simulink model "HexaMotor_LeadLag_Control_V03"  (R2026b)
settings: Solver=FixedStepDiscrete  StopTime=30  FixedStep=0.001  EnableMultiTasking=on
PreLoadFcn:
  | % HexaMotor custom Uno R4 blocks (Encoder Velocity, PWM, Analog Input) are
  | % System objects in the HexaMotorBlocks folder next to this model. Add it to
  | % the path if they aren't found (install_HexaMotor_V03 adds it permanently).
  | if ~exist('R4PWM', 'class') || ~exist('EncoderVelocity', 'class')
  |     addpath(fullfile(fileparts(get_param(bdroot, 'FileName')), 'HexaMotorBlocks'));
  |     if ~exist('R4PWM', 'class')
  |         warning('HexaMotor blocks not found. Run install_HexaMotor_V03 in the HexaMotor folder.');
  |     end
  | end
model workspace (MAT data in the model file):
  sampleRate = 0.001
libraries: simulink x2, eeGeneralControl x2, arduinolib x2, slpidlib x1
settings Model: SILPILModeSetting=veronly  Creator=bkhusain  LastModifiedBy=arkad
settings SolverCC: AutoInsertRateTranBlk=on
settings DataIOCC: DSMLogging=off  ReturnWorkspaceOutputs=off  SaveOutput=off  SaveTime=off
settings OptimizationCC: DifferentSizesBufferReuse=on  EnhancedBackFolding=on  MaxStackSize=64  OptimizationCustomize=off  OptimizeBlockOrder=speed
settings DebuggingCC: ParameterOverflowMsg=none  ParameterPrecisionLossMsg=none  ParameterTunabilityLossMsg=error  ParameterUnderflowMsg=error
settings HardwareCC: ProdHWDeviceType=ARM Compatible->ARM Cortex  ProdLargestAtomicFloat=Double  ProdLargestAtomicInteger=Long
settings SFSimCC: MATLABDynamicMemAlloc=off
settings RTWCC: BuildConfiguration=Faster Runs  DLArmComputeVersion=19.05  Description=Embedded Coder  HardwareBoard=Arduino Uno R4 Minima  SystemTargetFile=ert.tlc  TLCOptions=-aInlineSetEventsForThisBaseRateFcn=TLC_FALSE -aSuppressMultiTaskScheduler=TLC_FALSE -aRateBasedStepFcn=1  TemplateMakefile=ert_default_tmf  Toolchain=Arduino ARM M4
settings CodeAppCC: ForceParamTrailComments=on  OperatorAnnotations=on
settings ERTTargetCC: DynamicArrayContainerType=coder::array  ERTCustomFileBanners=off  ExtModeAutomaticAllocSize=off  ExtModeIntrfLevel=Level2 - Open  ExtModeMexFile=ext_xcp  ExtModeStaticAlloc=on  ModelStepFunctionPrototypeControlCompliant=off  SupportContinuousTime=on  SupportNonInlinedSFcns=on  SupportVariableSizeSignals=on
settings SimscapeCC: SimscapeUseEnergyAccounting=off

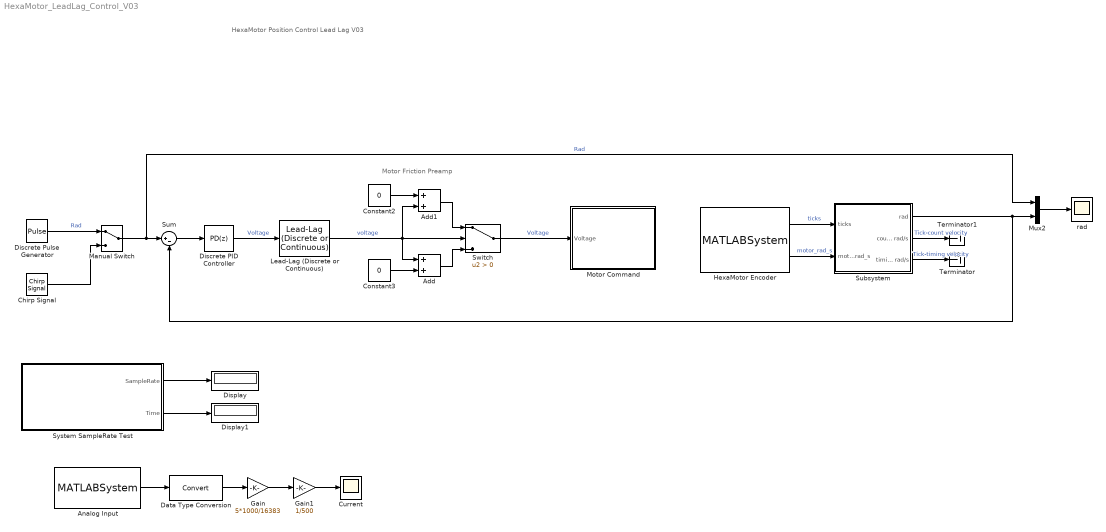
== system HexaMotor_LeadLag_Control_V03 ==
  note: HexaMotor
      | Position Control Lead Lag V03
  note: Motor Friction Preamp
  Add : Sum
  Add1 : Sum
  Analog Input : MATLABSystem  System=R4AnalogInput  Pin=A1  Reference=Default (AVCC, 5 V)  Resolution=14 bits  OutputType=Counts  ReferenceVoltage=5  SampleTime=-1
      mask Type: R4AnalogInput
  Chirp Signal : simulink/Sources/Chirp Signal  f1=0.1  T=30  f2=5
  Constant2 : Constant  Value=0  SampleTime=-1
  Constant3 : Constant  Value=0  SampleTime=-1
  Current : Scope
      settings: ActiveDisplayYMinimum=-0.12825795031435022  ActiveDisplayYMaximum=1.1543215528291522
  Data Type Conversion : DataTypeConversion  SaturateOnIntegerOverflow=off  RndMeth=Floor
  Discrete Pulse Generator : DiscretePulseGenerator  Period=4/sampleRate  PulseWidth=2/sampleRate  PhaseDelay=1/sampleRate  SampleTime=sampleRate
  Discrete PID Controller : slpidlib/PID Controller  Controller=PD  Form=Parallel  TimeDomain=Discrete-time  UseExternalTs=off  SampleTime=sampleRate  IntegratorMethod=Forward Euler  FilterMethod=Forward Euler  ControllerParametersSource=internal  P=10  I=5  UseKiTs=off  D=0  UseExternalDerivativeSource=off  N=100  UseFilter=on  TunerSelectOption=Transfer Function Based (PID Tuner App)  InitialConditionSource=internal  InitialConditionForIntegrator=0  InitialConditionForFilter=0  DifferentiatorICPrevScaledInput=0  ExternalReset=none  TrackingMode=off  Kt=1  LimitOutput=off  SatLimitsSource=internal  UpperSaturationLimit=inf  LowerSaturationLimit=-inf  LinearizeAsGain=off  AntiWindupMode=none  Kb=1  LimitIntegrator=off  UpperIntegratorSaturationLimit=inf  LowerIntegratorSaturationLimit=-inf  POutMin=[]  POutMax=[]  IOutMin=[]  IOutMax=[]  DOutMin=[]  DOutMax=[]  NOutMin=[]  NOutMax=[]  SumOutMin=[]  SumOutMax=[]  SaturationOutMin=[]  SaturationOutMax=[]  PParamMin=[]  PParamMax=[]  IParamMin=[]  IParamMax=[]  DParamMin=[]  DParamMax=[]  NParamMin=[]  NParamMax=[]  KbParamMin=[]  KbParamMax=[]  KtParamMin=[]  KtParamMax=[]  KbOutMin=[]  KbOutMax=[]  KtOutMin=[]  KtOutMax=[]  IntegratorOutMin=[]  IntegratorOutMax=[]  FilterOutMin=[]  FilterOutMax=[]  SumI1OutMin=[]  SumI1OutMax=[]  SumI2OutMin=[]  SumI2OutMax=[]  SumI3OutMin=[]  SumI3OutMax=[]  SumI4OutMin=[]  SumI4OutMax=[]  SumDOutMin=[]  SumDOutMax=[]  DifferentiatorOutMin=[]  DifferentiatorOutMax=[]  FilterDiffOutCoefMin=[]  FilterDiffOutCoefMax=[]  ReciprocalOutMin=[]  ReciprocalOutMax=[]  SumDenOutMin=[]  SumDenOutMax=[]  SumNumOutMin=[]  SumNumOutMax=[]  DivideOutMin=[]  DivideOutMax=[]  UdiffTsProdOutMin=[]  UdiffTsProdOutMax=[]  NTsProdOutMin=[]  NTsProdOutMax=[]  UintegralTsProdOutMin=[]  UintegralTsProdOutMax=[]  UngainTsProdOutMin=[]  UngainTsProdOutMax=[]  ClampingZeroOutDataTypeStr=Inherit: Inherit via back propagation  ClampingZeroOutMin=[]  ClampingZeroOutMax=[]  FilterDenConstantOutDataTypeStr=Inherit: Inherit via back propagation  FilterDenConstantOutMin=[]  FilterDenConstantOutMax=[]  PCopyOutDataTypeStr=Inherit: Inherit via back propagation  PCopyOutMin=[]  PCopyOutMax=[]  NCopyOutDataTypeStr=Inherit: Inherit via back propagation  NCopyOutMin=[]  NCopyOutMax=[]  IntegratorContinuousStateAttributes=''  IntegratorStateMustResolveToSignalObject=off  IntegratorRTWStateStorageClass=Auto  FilterContinuousStateAttributes=''  FilterStateMustResolveToSignalObject=off  FilterRTWStateStorageClass=Auto  ParallelPVariant=InternalParameters  IdealPVariant=Disabled  IVariant=Disabled  DVariant=InternalParameters  IntegratorVariant=Disabled  SatVariant=Disabled  AWVariant=Disabled  PCopyVariant=Disabled  TRVariant=Disabled  FdbkBlocksVariant=Forward  IdealPFdbkVariant=Disabled  SatFdbkVariant=Disabled  DerivativeFilterVariant=ForwardEulerFilter  NVariant=InternalParameters  NCopyVariant=Disabled  FilterICVariant=InternalICsFilter  IntegratorICVariant=Disabled  ExternalResetVariant=Disabled  TRSumVariant=Passthrough  SumFdbkVariant=Disabled  SumVariant=Sum_PD  TsampFilterVariant=InternalTs  TsampNgainVariant=Passthrough  TsampIntegralVariant=Disabled_SignalSpec  ExternalSaturationOutDataTypeStr=Inherit: Same as second input  DerivativeSourceVariant=ErrorSignal  PreIntVariant=InternalPreInt
      settings: LibrarySourceBlock=simulink/Discrete/Discrete PID Controller
  Display : Display
  Display1 : Display
  Gain : Gain  Gain=5*1000/16383
  Gain1 : Gain  Gain=1/500
  HexaMotor Encoder : MATLABSystem  Description=|  System=EncoderVelocity  PinA=2  PinB=3  EdgeMode=A and B both edges (4x)  PulsesPerRevolution=12  WindowLength=48  MaxWindowTime=0.01  StallTimeout=0.1  DecayWhenSlowing=on  DecayTolerance=1.5  CountAnchorTime=0.1  OutputFilterTime=0.005  Units=rad/s  OutputCount=on  TicksFirst=on  SampleTime=-1
      | HexaMotor Encoder (Encoder Velocity block, R4 Minima patch) - model V03_2
      | Outputs:
      |   ticks (int32): accumulated quadrature edge count, 4x decoding of the 12-line encoder on the motor shaft = 48 per motor turn = 979.2 per output turn.
      |   Motor_Rad/s (single): motor-shaft angular velocity in rad/s (before the 20.4:1 gearbox); the Subsystem divides by 20.4 for the output shaft.
      | Settings: 4x edges, window N <= 48 / 10 ms, decay tol 1.5, count anchor 0.1 s, output filter 2 ms, stall timeout 0.1 s, 1 kHz.
      mask Type: EncoderVelocity
  Lead-Lag (Discrete or Continuous) : eeGeneralControl/Lead-Lag (Discrete or Continuous)  T1=0  T2=0  B=inf  A=-inf  init_option=Inherited from block input  x0=0  Ts=-1
      settings: LibrarySourceBlock=|
      | ee_sl_lib/General Control/Lead-Lag
      | (Discrete or Continuous)
  Manual Switch : ManualSwitch
  Motor Command : Subsystem
  Mux2 : Mux  Inputs=2
  Subsystem : Subsystem
  Sum : Sum  Inputs=|+-
  Switch : Switch  Criteria=u2 > Threshold  SaturateOnIntegerOverflow=off  InputSameDT=off
  System SampleRate Test : Subsystem
  Terminator : Terminator
  Terminator1 : Terminator
  rad : Scope
      settings: ActiveDisplayYMinimum=-0.36735330763483587  ActiveDisplayYMaximum=1.3811842701903656
  wires:
  System SampleRate Test/1(SampleRate) -> Display/1
  System SampleRate Test/2(Time) -> Display1/1
  Sum/1 -> Discrete PID Controller/1
  Discrete Pulse Generator/1 -> Manual Switch/1  "Rad"
  Chirp Signal/1 -> Manual Switch/2
  Data Type Conversion/1 -> Gain/1
  Gain1/1 -> Current/1
  Gain/1 -> Gain1/1
  Constant3/1 -> Add/2
  Discrete PID Controller/1 -> Lead-Lag (Discrete or Continuous)/1  "Voltage"
  Constant2/1 -> Add1/1
  Add/1 -> Switch/3
  Manual Switch/1 -> Mux2/1, Sum/1  "Rad"
  Switch/1 -> Motor Command/1(Voltage)  "Voltage"
  Add1/1 -> Switch/1
  Subsystem/1(rad) -> Mux2/2, Sum/2
  Mux2/1 -> rad/1
  HexaMotor Encoder/1 -> Subsystem/1(ticks)  "ticks"
  HexaMotor Encoder/2 -> Subsystem/2(motor_rad_s)  "motor_rad_s"
  Subsystem/3(timing rad/s) -> Terminator/1  "Tick-timing velocity"
  Subsystem/2(count rad/s) -> Terminator1/1  "Tick-count velocity"
  Lead-Lag (Discrete or Continuous)/1 -> Add/1, Add1/2, Switch/2  "voltage"
  Analog Input/1 -> Data Type Conversion/1

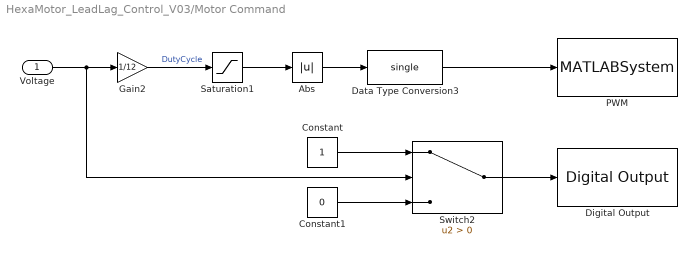
== system HexaMotor_LeadLag_Control_V03/Motor Command ==
  Voltage : Inport
  Abs : Abs  SaturateOnIntegerOverflow=off
  Constant : Constant  OutDataTypeStr=uint8  SampleTime=-1
  Constant1 : Constant  Value=0  OutDataTypeStr=uint8  SampleTime=-1
  Data Type Conversion3 : DataTypeConversion  OutDataTypeStr=single  SaturateOnIntegerOverflow=off  RndMeth=Floor
  Digital Output : arduinolib/Digital Output  pinNumber=8  Direction=output  blockPlatform=arduino
      settings: LibrarySourceBlock=gizmoLibrary/Arduino Utilities/Digital Output
  Gain2 : Gain  Gain=1/12
  PWM : MATLABSystem  System=R4PWM  Pin=10  DutyRange=0 to 1  FrequencySource=Parameter  Frequency=20000  MinFrequency=1000  OutputCounts=off  SampleTime=-1
      mask Type: R4PWM
  Saturation1 : Saturate  UpperLimit=1  LowerLimit=-1
  Switch2 : Switch  Criteria=u2 > Threshold  OutDataTypeStr=uint8  SaturateOnIntegerOverflow=off  InputSameDT=off
  wires:
  Voltage/1 -> Switch2/2, Gain2/1
  Abs/1 -> Data Type Conversion3/1
  Gain2/1 -> Saturation1/1  "DutyCycle"
  Constant1/1 -> Switch2/3
  Constant/1 -> Switch2/1
  Saturation1/1 -> Abs/1
  Switch2/1 -> Digital Output/1
  Data Type Conversion3/1 -> PWM/1

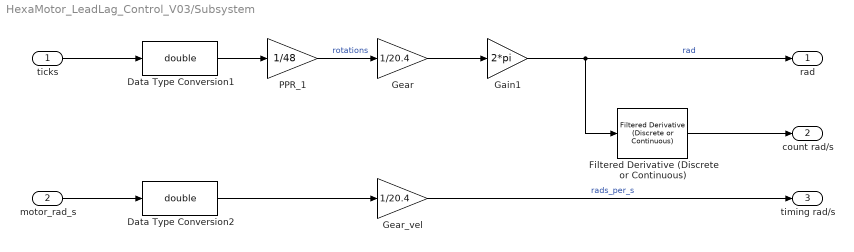
== system HexaMotor_LeadLag_Control_V03/Subsystem ==
  ticks : Inport
  motor_rad_s : Inport  Port=2
  Data Type Conversion1 : DataTypeConversion  OutDataTypeStr=double  SaturateOnIntegerOverflow=off  RndMeth=Floor
  Data Type Conversion2 : DataTypeConversion  OutDataTypeStr=double  SaturateOnIntegerOverflow=off  RndMeth=Floor
  Filtered Derivative (Discrete or Continuous) : eeGeneralControl/Filtered Derivative (Discrete or Continuous)  K=1  T=0.05  B=inf  A=-inf  minRatio=10  init_option=Inherited from block input  x0=0  Ts=-1
      settings: LibrarySourceBlock=|
      | ee_sl_lib/General Control/Filtered Derivative
      | (Discrete or Continuous)
  Gain1 : Gain  Gain=2*pi
  Gear : Gain  Gain=1/20.4
  Gear_vel : Gain  Gain=1/20.4
  PPR_1 : Gain  Gain=1/48
  rad : Outport
  count rad/s : Outport  Port=2
  timing rad/s : Outport  Port=3
  wires:
  PPR_1/1 -> Gear/1  "rotations"
  Data Type Conversion1/1 -> PPR_1/1
  ticks/1 -> Data Type Conversion1/1
  Gear/1 -> Gain1/1
  motor_rad_s/1 -> Data Type Conversion2/1
  Data Type Conversion2/1 -> Gear_vel/1
  Gain1/1 -> Filtered Derivative (Discrete or Continuous)/1, rad/1  "rad"
  Gear_vel/1 -> timing rad/s/1  "rads_per_s"
  Filtered Derivative (Discrete or Continuous)/1 -> count rad/s/1

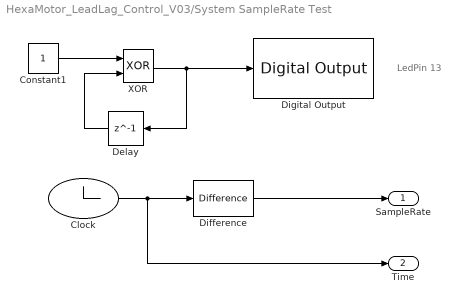
== system HexaMotor_LeadLag_Control_V03/System SampleRate Test ==
  note: LedPin 13
  Clock : Clock
      settings: Decimation=3
  Constant1 : Constant  SampleTime=-1
  Delay : Delay  DelayLength=1  InitialCondition=0
  Difference : simulink/Quick Insert/Discrete/Difference  ICPrevInput=0.0  OutMin=[]  OutMax=[]  OutDataType=fixdt(1, 16)  OutScaling=2^-10  DoSatur=off
  Digital Output : arduinolib/Digital Output  pinNumber=13  Direction=output  blockPlatform=arduino
  XOR : Logic  Operator=XOR  IconShape=distinctive  AllPortsSameDT=off  OutDataTypeStr=boolean
  SampleRate : Outport
  Time : Outport  Port=2
  wires:
  XOR/1 -> Digital Output/1, Delay/1
  Constant1/1 -> XOR/1
  Delay/1 -> XOR/2
  Clock/1 -> Time/1, Difference/1
  Difference/1 -> SampleRate/1
